simulink subsystem "Sensors"  (R2024b)
settings: Solver=VariableStepAuto  StartTime=0.0  StopTime=10.0  RelTol=1e-3
undefined symbols (not defined in the file): actuators, spacecraft
libraries: vrlib x8, sadlib x5, matrix_library x2
settings Model: Creator=marco  LastModifiedBy=domac

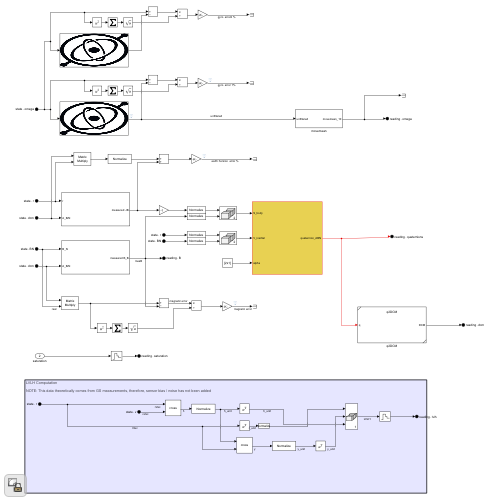
[thumbnail: Simulink's stored preview of the top-level diagram]
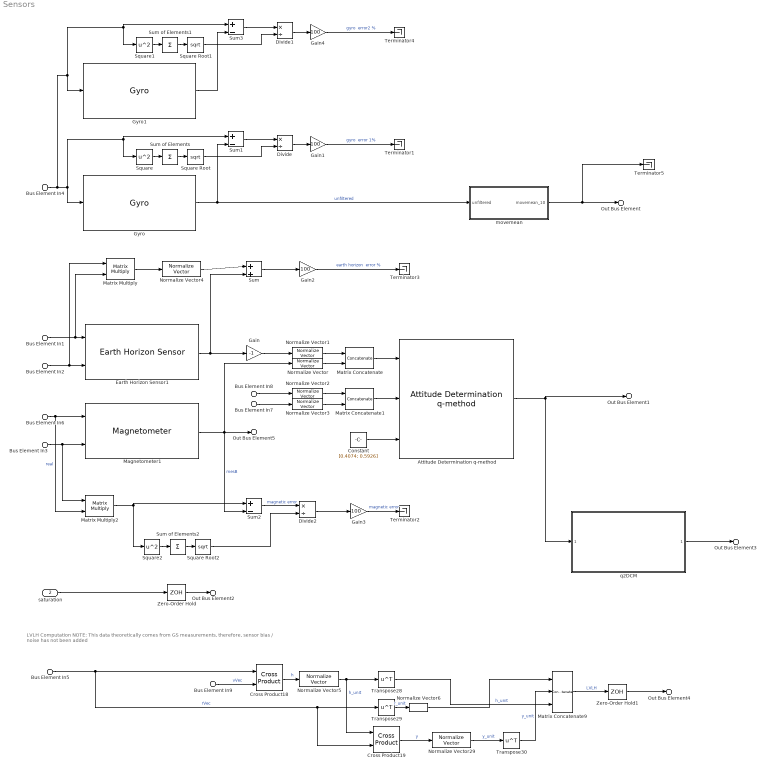
== system Sensors ==
  note: LVLH Computation
      |
      | NOTE: This data theoretically comes from GS measurements, therefore, sensor bias / noise has not been added
  Bus Element In2 : Inport  PortName=state  Element=dcm
  Bus Element In3 : Inport  PortName=state  Element=dcm
  Bus Element In4 : Inport  PortName=state  Element=omega
  Bus Element In1 : Inport  PortName=state  Element=r
  Bus Element In8 : Inport  PortName=state  Element=r
  Bus Element In5 : Inport  PortName=state  Element=r
  Bus Element In9 : Inport  PortName=state  Element=v
  Bus Element In6 : Inport  PortName=state  Element=BN
  Bus Element In7 : Inport  PortName=state  Element=BN
  saturation : Inport  Port=2
  Attitude Determination q-method : sadlib/Attitude Determination q-method  SystemSampleTime=-1  VariantActivationTime=update diagram  AllowFlexibleInterface=on  Latency=0  AutoFrameSizeCalculation=off
  Constant : Constant  Value=[0.4074; 0.5926]
  Cross Product18 : matrix_library/Cross Product
  Cross Product19 : matrix_library/Cross Product
  Divide : Product  Inputs=*/
  Divide1 : Product  Inputs=*/
  Divide2 : Product  Inputs=*/
  Earth Horizon Sensor1 : sadlib/Earth Horizon Sensor  horizon=spacecraft.sensors.horizon  seed=spacecraft.sensors.horizon.seed
  Gain : Gain  Gain=-1
  Gain{1..4} (4 alike) : Gain  Gain=100
  Gyro : sadlib/Gyro  gyro=spacecraft.sensors.gyro(1)  seed=spacecraft.sensors.gyro(1).seed
  Gyro1 : sadlib/Gyro  gyro=spacecraft.sensors.gyro(2)  seed=spacecraft.sensors.gyro(2).seed
  Magnetometer1 : sadlib/Magnetometer  magneto=spacecraft.sensors.magnetometer  seed=spacecraft.sensors.magnetometer.seed
  Matrix Concatenate : Concatenate  Mode=Multidimensional array  ConcatenateDimension=2
  Matrix Concatenate1 : Concatenate  Mode=Multidimensional array  ConcatenateDimension=2
  Matrix Concatenate9 : Concatenate  NumInputs=3  Mode=Multidimensional array
  Matrix Multiply : Product  Multiplication=Matrix(*)
  Matrix Multiply2 : Product  Multiplication=Matrix(*)
  Normalize Vector{,1..6,29} (8 alike) : vrlib/Utilities/Normalize Vector  maxzero=0
  Square : Math  Operator=square
  Square Root : Sqrt
  Square Root1 : Sqrt
  Square Root2 : Sqrt
  Square1 : Math  Operator=square
  Square2 : Math  Operator=square
  Sum : Sum  Inputs=|++
  Sum of Elements : Sum  Inputs=+
  Sum of Elements1 : Sum  Inputs=+
  Sum of Elements2 : Sum  Inputs=+
  Sum1 : Sum  Inputs=|+-
  Sum2 : Sum  Inputs=|+-
  Sum3 : Sum  Inputs=|+-
  Terminator{1..5} (5 alike) : Terminator
  Transpose28 : Math  Operator=transpose
  Transpose29 : Math  Operator=transpose
  Transpose30 : Math  Operator=transpose
  Zero-Order Hold : ZeroOrderHold  SampleTime=actuators.wheel.sT
  Zero-Order Hold1 : ZeroOrderHold  SampleTime=0.01
  movemean : Subsystem
  q2DCM : Subsystem  ReferencedSubsystem=q2DCM
  Out Bus Element : Outport  PortName=reading  Element=omega
  Out Bus Element1 : Outport  PortName=reading  Element=quaternions
  Out Bus Element2 : Outport  PortName=reading  Element=saturation
  Out Bus Element3 : Outport  PortName=reading  Element=dcm
  Out Bus Element4 : Outport  PortName=reading  Element=lvlh
  Out Bus Element5 : Outport  PortName=reading  Element=B
  wires:
  Normalize Vector/1 -> Matrix Concatenate/2
  Matrix Concatenate/1 -> Attitude Determination q-method/1
  Constant/1 -> Attitude Determination q-method/3
  Bus Element In1/1 -> Earth Horizon Sensor1/1, Matrix Multiply/2
  Gain/1 -> Normalize Vector1/1
  Earth Horizon Sensor1/1 -> Gain/1, Sum/2
  Bus Element In2/1 -> Earth Horizon Sensor1/2, Matrix Multiply/1
  Normalize Vector3/1 -> Matrix Concatenate1/2
  Normalize Vector1/1 -> Matrix Concatenate/1
  Normalize Vector2/1 -> Matrix Concatenate1/1
  Magnetometer1/1 -> Normalize Vector/1, Out Bus Element5/1, Sum2/2  "mesB"
  Matrix Concatenate1/1 -> Attitude Determination q-method/2
  Attitude Determination q-method/1 -> Out Bus Element1/1, q2DCM/1
  Gyro/1 -> Sum1/2, movemean/1(unfiltered)  "unfiltered"
  Bus Element In3/1 -> Magnetometer1/2, Matrix Multiply2/1
  Bus Element In7/1 -> Normalize Vector3/1
  Bus Element In8/1 -> Normalize Vector2/1
  saturation/1 -> Zero-Order Hold/1
  Matrix Multiply/1 -> Normalize Vector4/1
  Gain3/1 -> Terminator2/1  "magnetic error"
  Matrix Multiply2/1 -> Sum2/1, Square2/1
  Square/1 -> Sum of Elements/1
  Sum of Elements/1 -> Square Root/1
  Sum1/1 -> Divide/1
  Square Root/1 -> Divide/2
  Divide/1 -> Gain1/1
  Gain1/1 -> Terminator1/1  "gyro  error 1%"
  Gain2/1 -> Terminator3/1  "earth horizon  error %"
  Sum/1 -> Gain2/1
  Divide2/1 -> Gain3/1
  Sum2/1 -> Divide2/1  "magnetic error"
  Square2/1 -> Sum of Elements2/1
  Sum of Elements2/1 -> Square Root2/1
  Square Root2/1 -> Divide2/2
  Bus Element In6/1 -> Magnetometer1/1, Matrix Multiply2/2  "real"
  Normalize Vector4/1 -> Sum/1
  Gain4/1 -> Terminator4/1  "gyro  error2 %"
  Divide1/1 -> Gain4/1
  Square Root1/1 -> Divide1/2
  Sum3/1 -> Divide1/1
  Sum of Elements1/1 -> Square Root1/1
  Square1/1 -> Sum of Elements1/1
  Bus Element In4/1 -> Gyro/1, Sum1/1, Square/1, Square1/1, Sum3/1, Gyro1/1
  Gyro1/1 -> Sum3/2
  Transpose28/1 -> Matrix Concatenate9/3  "h_unit"
  Transpose29/1 -> Normalize Vector6/1  "r_unit"
  Matrix Concatenate9/1 -> Zero-Order Hold1/1  "LVLH"
  Bus Element In5/1 -> Cross Product18/1, Cross Product19/2, Transpose29/1  "rVec"
  Normalize Vector29/1 -> Transpose30/1  "y_unit"
  Bus Element In9/1 -> Cross Product18/2  "vVec"
  Cross Product19/1 -> Normalize Vector29/1  "y"
  Cross Product18/1 -> Normalize Vector5/1  "h"
  Normalize Vector5/1 -> Cross Product19/1, Transpose28/1  "h_unit"
  Transpose30/1 -> Matrix Concatenate9/2  "y_unit"
  Normalize Vector6/1 -> Matrix Concatenate9/1
  Zero-Order Hold/1 -> Out Bus Element2/1
  Zero-Order Hold1/1 -> Out Bus Element4/1
  movemean/1(movemean_10) -> Terminator5/1, Out Bus Element/1
  q2DCM/1 -> Out Bus Element3/1

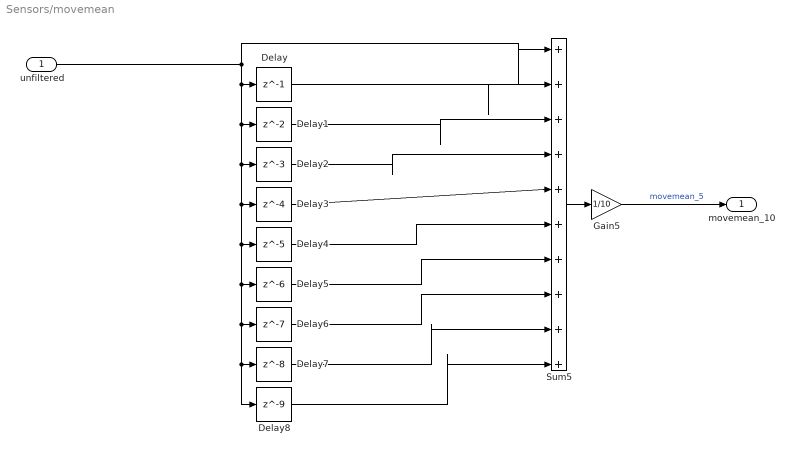
== system Sensors/movemean ==
  unfiltered : Inport
  Delay : Delay  DelayLength=1
  Delay1 : Delay
  Delay2 : Delay  DelayLength=3
  Delay3 : Delay  DelayLength=4
  Delay4 : Delay  DelayLength=5
  Delay5 : Delay  DelayLength=6
  Delay6 : Delay  DelayLength=7
  Delay7 : Delay  DelayLength=8
  Delay8 : Delay  DelayLength=9
  Gain5 : Gain  Gain=1/10
  Sum5 : Sum  Inputs=|++++++++++
  movemean_10 : Outport
  wires:
  Gain5/1 -> movemean_10/1  "movemean_5"
  Sum5/1 -> Gain5/1
  Delay6/1 -> Sum5/8
  Delay8/1 -> Sum5/10
  Delay5/1 -> Sum5/7
  Delay2/1 -> Sum5/4
  Delay7/1 -> Sum5/9
  Delay/1 -> Sum5/2
  Delay4/1 -> Sum5/6
  Delay3/1 -> Sum5/5
  unfiltered/1 -> Delay/1, Delay1/1, Delay2/1, Delay3/1, Delay4/1, Delay5/1, Delay6/1, Delay7/1, Delay8/1, Sum5/1
  Delay1/1 -> Sum5/3
